simulink library "cntrlPosNdi_lib"  (R2018b)
settings: Solver=VariableStepAuto  StartTime=0.0  StopTime=10.0  RelTol=1e-3
undefined symbols (not defined in the file or in its folder): DiscIntNeverNeededParam, psc
libraries: simulink x2, $bdroot x2
settings Model: Creator=Ybeyer  LastModifiedBy=yannic
settings SFSimCC: SimUseLocalCustomCode=off
settings RTWCC: RTWUseLocalCustomCode=off
settings CodeAppCC: StateflowObjectComments=on

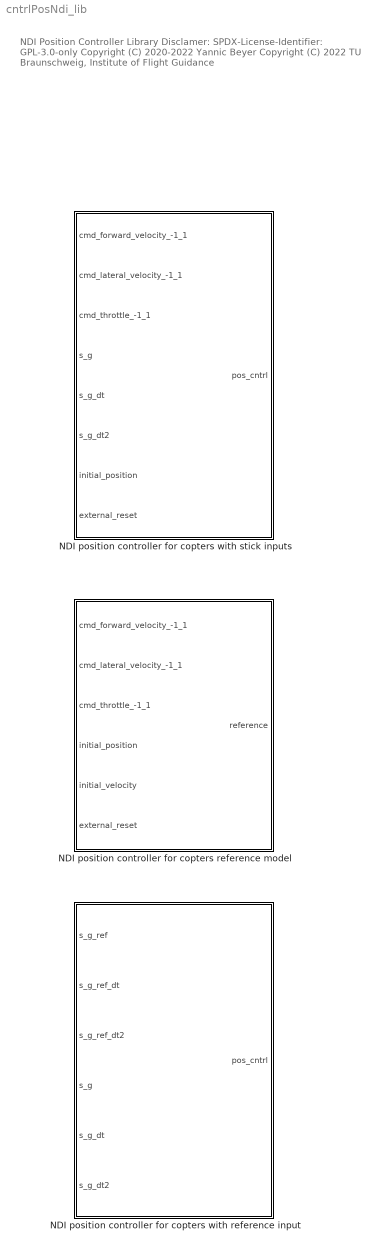
== system cntrlPosNdi_lib ==
  note: NDI Position Controller Library
      |
      | Disclamer:
      | SPDX-License-Identifier: GPL-3.0-only
      |
      | Copyright (C) 2020-2022 Yannic Beyer
      | Copyright (C) 2022 TU Braunschweig, Institute of Flight Guidance
  NDI position controller for copters reference model : Subsystem  mask{psc=psc, is_enable_checked=off, states_when_enabling=held}
      mask prompts: psc "position controller parameters struct, see cntrlPosIndi_params_default"; is_enable_checked "Activate "Enabled Subsystem""; states_when_enabling "States when enabling:"
      mask init:
      | cntrlBlockInit(is_enable_checked,states_when_enabling);
      mask TypeOptions states_when_enabling: held | reset
      mask DialogControl DescGroupVar Prompt: NDI position controller for copters reference model
      mask DialogControl DescTextVar Prompt: The commanded velocity is filtered and reference signals are generated.
  NDI position controller for copters with reference input : Subsystem  mask{psc=psc, T_inner_loop=0.1, is_enable_checked=off, states_when_enabling=held}
      mask prompts: psc "Position controller parameters struct, see cntrlPosIndi_params_default"; T_inner_loop "Inner loop time constant, in s"; is_enable_checked "Activate "Enabled Subsystem""; states_when_enabling "States when enabling:"
      mask init:
      | cntrlBlockInit(is_enable_checked,states_when_enabling);
      mask TypeOptions states_when_enabling: held | reset
      mask DialogControl DescGroupVar Prompt: NDI position controller cascade with reference inputs
      mask DialogControl DescTextVar Prompt: The controller takes reference signals as input and the control error is converted into desired accerlations.
  NDI position controller for copters with stick inputs : Subsystem  mask{psc=psc, T_inner_loop=0.1, is_enable_checked=off, states_when_enabling=held}
      mask prompts: psc "position controller parameters struct, see cntrlPosIndi_params_default"; T_inner_loop "inner loop time constant, in s"; is_enable_checked "Activate "Enabled Subsystem""; states_when_enabling "States when enabling:"
      mask init:
      | cntrlBlockInit(is_enable_checked,states_when_enabling);
      mask TypeOptions states_when_enabling: held | reset
      mask DialogControl DescGroupVar Prompt: NDI Position controller cascade
      mask DialogControl DescTextVar Prompt: The commanded velocity is filtered and the control error is converted into desired accerlations.

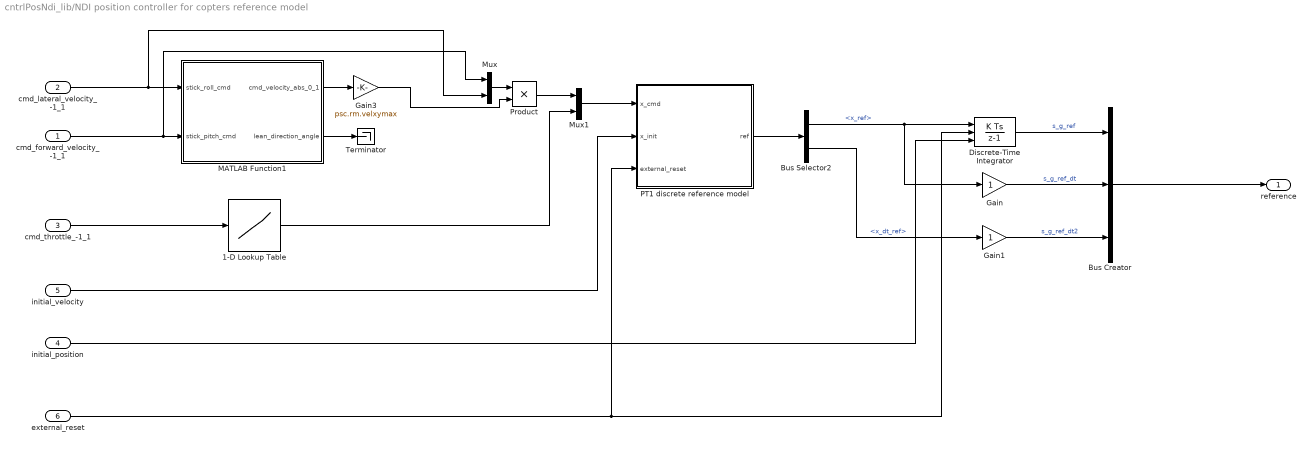
== system cntrlPosNdi_lib/NDI position controller for copters reference model ==
  cmd_forward_velocity_-1_1 : Inport
  cmd_lateral_velocity_-1_1 : Inport  Port=2
  cmd_throttle_-1_1 : Inport  Port=3
  initial_position : Inport  Port=4
  initial_velocity : Inport  Port=5
  external_reset : Inport  Port=6
  1-D Lookup Table : Lookup_n-D  NumberOfTableDimensions=1  BreakpointsForDimension1=[-1,0,1]  Table=[psc.rm.veldmax,0,-psc.rm.velumax]  InternalRulePriority=Speed  RndMeth=Simplest  InputSameDT=on
  Bus Creator : BusCreator  Inputs=3
  Bus Selector2 : BusSelector  OutputSignals=x_ref,x_dt_ref
  Discrete-Time Integrator : DiscreteIntegrator  ExternalReset=rising  InitialConditionSource=external  SampleTime=-1  ICPrevOutput=DiscIntNeverNeededParam  ICPrevScaledInput=DiscIntNeverNeededParam
  Gain : Gain
  Gain1 : Gain
  Gain3 : Gain  Gain=psc.rm.velxymax
  MATLAB Function1 : MATLAB Function  TreatAsAtomicUnit=on
  Mux : Mux  Inputs=2
  Mux1 : Mux  Inputs=2
  PT1 discrete reference model : Subsystem  mask{T=psc.rm.veltc, x_max=inf, x_min=-inf, x_dt_max=[psc.rm.accxymax*[1;1]; psc.rm.accdmax], x_dt_min=[-psc.rm.accxymax*[1;1]; -psc.rm.accumax], x_init=0}
      mask prompts: T "Time constant"; x_max "Maximum position"; x_min "Minimum position"; x_dt_max "Maximum rate"; x_dt_min "Minimum rate"; x_init "Initial position"
  Product : Product
  Terminator : Terminator
  reference : Outport
  wires:
  cmd_forward_velocity_-1_1/1 -> Mux/1, MATLAB Function1/2(stick_pitch_cmd)
  Bus Creator/1 -> reference/1
  PT1 discrete reference model/1(ref) -> Bus Selector2/1
  Discrete-Time Integrator/1 -> Bus Creator/1  "s_g_ref"
  Bus Selector2/1 -> Gain/1, Discrete-Time Integrator/1  "<x_ref>"
  Bus Selector2/2 -> Gain1/1  "<x_dt_ref>"
  cmd_lateral_velocity_-1_1/1 -> Mux/2, MATLAB Function1/1(stick_roll_cmd)
  Gain/1 -> Bus Creator/2  "s_g_ref_dt"
  Gain1/1 -> Bus Creator/3  "s_g_ref_dt2"
  Mux/1 -> Product/1
  MATLAB Function1/2(lean_direction_angle) -> Terminator/1
  MATLAB Function1/1(cmd_velocity_abs_0_1) -> Gain3/1
  Product/1 -> Mux1/1
  Gain3/1 -> Product/2
  cmd_throttle_-1_1/1 -> 1-D Lookup Table/1
  Mux1/1 -> PT1 discrete reference model/1(x_cmd)
  1-D Lookup Table/1 -> Mux1/2
  external_reset/1 -> PT1 discrete reference model/3(external_reset), Discrete-Time Integrator/2
  initial_position/1 -> Discrete-Time Integrator/3
  initial_velocity/1 -> PT1 discrete reference model/2(x_init)

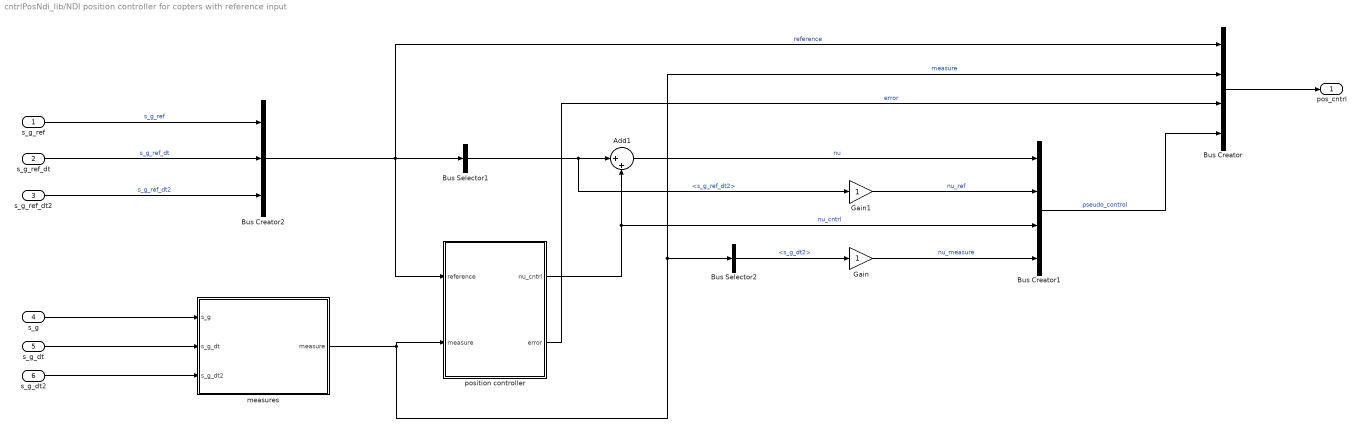
== system cntrlPosNdi_lib/NDI position controller for copters with reference input ==
  s_g_ref : Inport
  s_g_ref_dt : Inport  Port=2
  s_g_ref_dt2 : Inport  Port=3
  s_g : Inport  Port=4
  s_g_dt : Inport  Port=5
  s_g_dt2 : Inport  Port=6
  Add1 : Sum  Inputs=|++
  Bus Creator : BusCreator  Inputs=4
  Bus Creator1 : BusCreator  Inputs=4
  Bus Creator2 : BusCreator  Inputs=3
  Bus Selector1 : BusSelector  OutputSignals=s_g_ref_dt2
  Bus Selector2 : BusSelector  OutputSignals=s_g_dt2
  Gain : Gain
  Gain1 : Gain
  measures : Subsystem
  position controller : Subsystem
  pos_cntrl : Outport
  wires:
  Bus Creator2/1 -> Bus Creator/1, position controller/1(reference), Bus Selector1/1  "reference"
  position controller/1(nu_cntrl) -> Add1/2, Bus Creator1/3  "nu_cntrl"
  Add1/1 -> Bus Creator1/1  "nu"
  s_g_dt2/1 -> measures/3(s_g_dt2)
  position controller/2(error) -> Bus Creator/3  "error"
  s_g/1 -> measures/1(s_g)
  s_g_dt/1 -> measures/2(s_g_dt)
  measures/1(measure) -> position controller/2(measure), Bus Selector2/1, Bus Creator/2  "measure"
  Bus Creator1/1 -> Bus Creator/4  "pseudo_control"
  Bus Creator/1 -> pos_cntrl/1
  Gain/1 -> Bus Creator1/4  "nu_measure"
  Bus Selector1/1 -> Gain1/1, Add1/1  "<s_g_ref_dt2>"
  Gain1/1 -> Bus Creator1/2  "nu_ref"
  s_g_ref/1 -> Bus Creator2/1  "s_g_ref"
  s_g_ref_dt/1 -> Bus Creator2/2  "s_g_ref_dt"
  s_g_ref_dt2/1 -> Bus Creator2/3  "s_g_ref_dt2"
  Bus Selector2/1 -> Gain/1  "<s_g_dt2>"

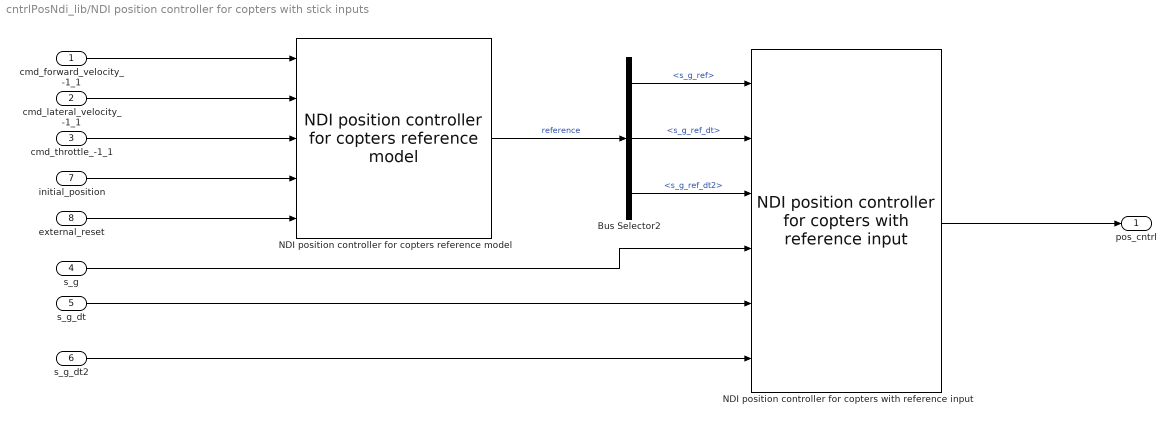
== system cntrlPosNdi_lib/NDI position controller for copters with stick inputs ==
  cmd_forward_velocity_-1_1 : Inport
  cmd_lateral_velocity_-1_1 : Inport  Port=2
  cmd_throttle_-1_1 : Inport  Port=3
  s_g : Inport  Port=4
  s_g_dt : Inport  Port=5
  s_g_dt2 : Inport  Port=6
  initial_position : Inport  Port=7
  external_reset : Inport  Port=8
  Bus Selector2 : BusSelector  OutputSignals=s_g_ref,s_g_ref_dt,s_g_ref_dt2
  NDI position controller for copters reference model : $bdroot/NDI position controller for copters reference model  psc=psc  is_enable_checked=off  states_when_enabling=held
  NDI position controller for copters with reference input : $bdroot/NDI position controller for copters with reference input  psc=psc  T_inner_loop=T_inner_loop  is_enable_checked=off  states_when_enabling=held
  pos_cntrl : Outport
  wires:
  cmd_forward_velocity_-1_1/1 -> NDI position controller for copters reference model/1
  initial_position/1 -> NDI position controller for copters reference model/4
  s_g_dt2/1 -> NDI position controller for copters with reference input/6
  s_g/1 -> NDI position controller for copters with reference input/4
  s_g_dt/1 -> NDI position controller for copters with reference input/5
  cmd_lateral_velocity_-1_1/1 -> NDI position controller for copters reference model/2
  cmd_throttle_-1_1/1 -> NDI position controller for copters reference model/3
  NDI position controller for copters reference model/1 -> Bus Selector2/1  "reference"
  Bus Selector2/1 -> NDI position controller for copters with reference input/1  "<s_g_ref>"
  Bus Selector2/2 -> NDI position controller for copters with reference input/2  "<s_g_ref_dt>"
  Bus Selector2/3 -> NDI position controller for copters with reference input/3  "<s_g_ref_dt2>"
  NDI position controller for copters with reference input/1 -> pos_cntrl/1
  external_reset/1 -> NDI position controller for copters reference model/5

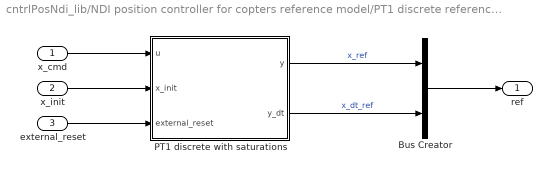
== system cntrlPosNdi_lib/NDI position controller for copters reference model/PT1 discrete reference model ==
  x_cmd : Inport
  x_init : Inport  Port=2
  external_reset : Inport  Port=3
  Bus Creator : BusCreator  Inputs=2
  PT1 discrete with saturations : Subsystem  mask{T=T, x_max=x_max, x_min=x_min, x_dt_max=x_dt_max, x_dt_min=x_dt_min, x_init=x_init}
      mask prompts: T "Time constant"; x_max "Maximum output"; x_min "Minimum output"; x_dt_max "Maximum output rate"; x_dt_min "Minimum output rate"; x_init "Initial output"
  ref : Outport
  wires:
  x_cmd/1 -> PT1 discrete with saturations/1(u)
  Bus Creator/1 -> ref/1
  PT1 discrete with saturations/1(y) -> Bus Creator/1  "x_ref"
  PT1 discrete with saturations/2(y_dt) -> Bus Creator/2  "x_dt_ref"
  external_reset/1 -> PT1 discrete with saturations/3(external_reset)
  x_init/1 -> PT1 discrete with saturations/2(x_init)

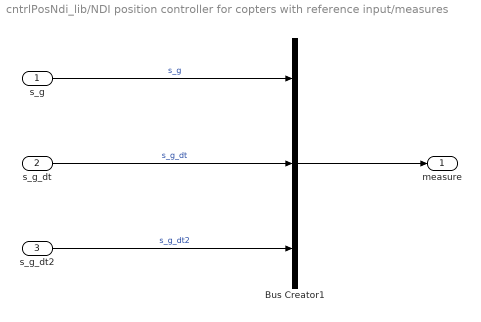
== system cntrlPosNdi_lib/NDI position controller for copters with reference input/measures ==
  s_g : Inport
  s_g_dt : Inport  Port=2
  s_g_dt2 : Inport  Port=3
  Bus Creator1 : BusCreator  Inputs=3
  measure : Outport
  wires:
  Bus Creator1/1 -> measure/1
  s_g_dt2/1 -> Bus Creator1/3  "s_g_dt2"
  s_g/1 -> Bus Creator1/1  "s_g"
  s_g_dt/1 -> Bus Creator1/2  "s_g_dt"

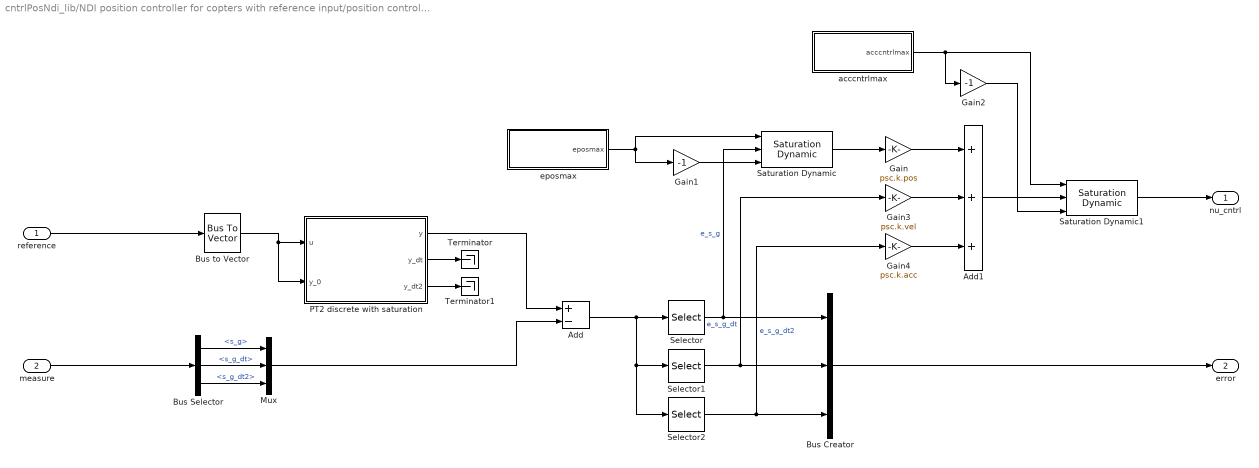
== system cntrlPosNdi_lib/NDI position controller for copters with reference input/position controller ==
  reference : Inport
  measure : Inport  Port=2
  Add : Sum  Inputs=+-
  Add1 : Sum  Inputs=+++
  Bus Creator : BusCreator  Inputs=3
  Bus Selector : BusSelector  OutputSignals=s_g,s_g_dt,s_g_dt2
  Bus to Vector : BusToVector
  Gain : Gain  Gain=psc.k.pos
  Gain1 : Gain  Gain=-1
  Gain2 : Gain  Gain=-1
  Gain3 : Gain  Gain=psc.k.vel
  Gain4 : Gain  Gain=psc.k.acc
  Mux : Mux  Inputs=3
  PT2 discrete with saturation : Subsystem  mask{omega=2./T_inner_loop, d=1, x_dt2_max=inf, x_dt2_min=-inf, x_dt_max=inf, x_dt_min=-inf, x_max=inf, x_min=-inf, x_init=0, x_dt_init=0}
      mask prompts: omega "Natural frequency"; d "Damping ratio"; x_dt2_max "Maximum acceleration"; x_dt2_min "Minimum acceleration"; x_dt_max "Maximum rate"; x_dt_min "Minimum rate"; x_max "Maximum position"; x_min "Minimum position"; x_init "Initial position"; x_dt_init "Initial rate"
  Saturation Dynamic : simulink/Discontinuities/Saturation Dynamic  OutMin=[]  OutMax=[]  OutDataTypeStr=Inherit: Same as second input  OutDataType=fixdt(1, 16)  OutScaling=2^-10  DoSatur=off
  Saturation Dynamic1 : simulink/Discontinuities/Saturation Dynamic  OutMin=[]  OutMax=[]  OutDataTypeStr=Inherit: Same as second input  OutDataType=fixdt(1, 16)  OutScaling=2^-10  DoSatur=off
  Selector : Selector  InputPortWidth=9  IndexOptions=Index vector (dialog)  Indices=1:3  OutputSizes=1
  Selector1 : Selector  InputPortWidth=9  IndexOptions=Index vector (dialog)  Indices=4:6  OutputSizes=1
  Selector2 : Selector  InputPortWidth=9  IndexOptions=Index vector (dialog)  Indices=7:9  OutputSizes=1
  Terminator : Terminator
  Terminator1 : Terminator
  acccntrlmax : MATLAB Function  TreatAsAtomicUnit=on
  eposmax : MATLAB Function  TreatAsAtomicUnit=on
  nu_cntrl : Outport
  error : Outport  Port=2
  wires:
  reference/1 -> Bus to Vector/1
  Add/1 -> Selector2/1, Selector1/1, Selector/1
  Saturation Dynamic1/1 -> nu_cntrl/1
  Add1/1 -> Saturation Dynamic1/2
  measure/1 -> Bus Selector/1
  Mux/1 -> Add/2
  Bus Selector/3 -> Mux/3  "<s_g_dt2>"
  Bus Selector/2 -> Mux/2  "<s_g_dt>"
  Bus Selector/1 -> Mux/1  "<s_g>"
  Bus to Vector/1 -> PT2 discrete with saturation/2(y_0), PT2 discrete with saturation/1(u)
  PT2 discrete with saturation/2(y_dt) -> Terminator/1
  PT2 discrete with saturation/3(y_dt2) -> Terminator1/1
  PT2 discrete with saturation/1(y) -> Add/1
  Selector/1 -> Saturation Dynamic/2, Bus Creator/1  "e_s_g"
  Selector1/1 -> Bus Creator/2, Gain3/1  "e_s_g_dt"
  Selector2/1 -> Gain4/1, Bus Creator/3  "e_s_g_dt2"
  Bus Creator/1 -> error/1
  eposmax/1(eposmax) -> Saturation Dynamic/1, Gain1/1
  Gain1/1 -> Saturation Dynamic/3
  acccntrlmax/1(acccntrlmax) -> Saturation Dynamic1/1, Gain2/1
  Gain2/1 -> Saturation Dynamic1/3
  Gain/1 -> Add1/1
  Gain3/1 -> Add1/2
  Gain4/1 -> Add1/3
  Saturation Dynamic/1 -> Gain/1

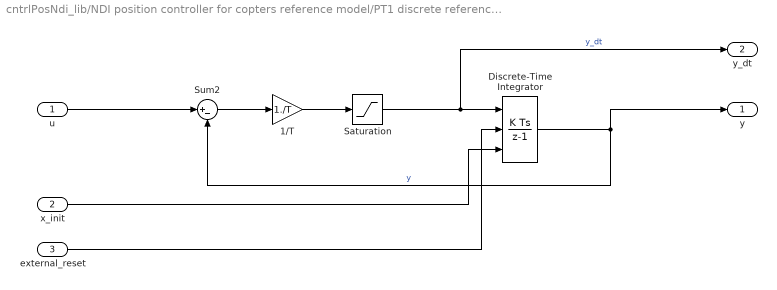
== system cntrlPosNdi_lib/NDI position controller for copters reference model/PT1 discrete reference model/PT1 discrete with saturations ==
  u : Inport
  x_init : Inport  Port=2
  external_reset : Inport  Port=3
  1/T : Gain  Gain=1./T
  Discrete-Time Integrator : DiscreteIntegrator  ExternalReset=rising  InitialConditionSource=external  InitialCondition=x_init  SampleTime=-1  LimitOutput=on  UpperSaturationLimit=x_max  LowerSaturationLimit=x_min  ICPrevOutput=DiscIntNeverNeededParam  ICPrevScaledInput=DiscIntNeverNeededParam
  Saturation : Saturate  UpperLimit=x_dt_max  LowerLimit=x_dt_min
  Sum2 : Sum  Inputs=|+-
  y : Outport
  y_dt : Outport  Port=2
  wires:
  1/T/1 -> Saturation/1
  u/1 -> Sum2/1
  Sum2/1 -> 1/T/1
  Discrete-Time Integrator/1 -> y/1, Sum2/2  "y"
  Saturation/1 -> Discrete-Time Integrator/1, y_dt/1  "y_dt"
  external_reset/1 -> Discrete-Time Integrator/2
  x_init/1 -> Discrete-Time Integrator/3

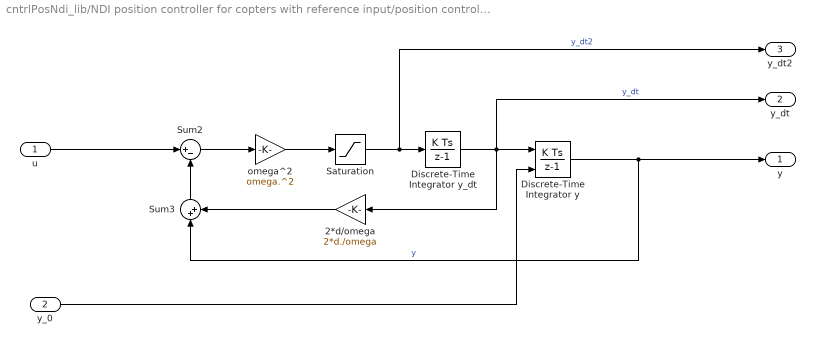
== system cntrlPosNdi_lib/NDI position controller for copters with reference input/position controller/PT2 discrete with saturation ==
  u : Inport
  y_0 : Inport  Port=2
  2*d/omega : Gain  Gain=2*d./omega
  Discrete-Time Integrator y : DiscreteIntegrator  InitialConditionSource=external  InitialCondition=x_init  SampleTime=-1  LimitOutput=on  UpperSaturationLimit=x_max  LowerSaturationLimit=x_min  ICPrevOutput=DiscIntNeverNeededParam  ICPrevScaledInput=DiscIntNeverNeededParam
  Discrete-Time Integrator y_dt : DiscreteIntegrator  InitialCondition=x_dt_init  SampleTime=-1  LimitOutput=on  UpperSaturationLimit=x_dt_max  LowerSaturationLimit=x_dt_min  ICPrevOutput=DiscIntNeverNeededParam  ICPrevScaledInput=DiscIntNeverNeededParam
  Saturation : Saturate  UpperLimit=x_dt2_max  LowerLimit=x_dt2_min
  Sum2 : Sum  Inputs=|+-
  Sum3 : Sum  Inputs=|++
  omega^2 : Gain  Gain=omega.^2
  y : Outport
  y_dt : Outport  Port=2
  y_dt2 : Outport  Port=3
  wires:
  Saturation/1 -> y_dt2/1, Discrete-Time Integrator y_dt/1  "y_dt2"
  omega^2/1 -> Saturation/1
  Sum3/1 -> Sum2/2
  u/1 -> Sum2/1
  2*d/omega/1 -> Sum3/2
  Sum2/1 -> omega^2/1
  Discrete-Time Integrator y/1 -> Sum3/1, y/1  "y"
  Discrete-Time Integrator y_dt/1 -> 2*d/omega/1, y_dt/1, Discrete-Time Integrator y/1  "y_dt"
  y_0/1 -> Discrete-Time Integrator y/2

== matlab function cntrlPosNdi_lib/NDI position controller for copters reference model/MATLAB Function1 ==
  data: stick_roll_cmd input; cmd_velocity_abs_0_1 output; stick_pitch_cmd input; lean_direction_angle output
function [cmd_velocity_abs_0_1,lean_direction_angle] = fcn(stick_roll_cmd,stick_pitch_cmd)

lean_direction_angle = atan2(stick_roll_cmd,-stick_pitch_cmd);
cmd_velocity_abs_0_1 = sqrt( stick_roll_cmd^2 + stick_pitch_cmd^2 );

end

== matlab function cntrlPosNdi_lib/NDI position controller for copters with reference input/position controller/eposmax ==
  data: eposmax output; psc parameter
function eposmax = fcn(psc)
eposmax = abs( divideFinite( psc.k.vel * psc.rm.velxymax * 0.7, psc.k.pos ) );
end

== matlab function cntrlPosNdi_lib/NDI position controller for copters with reference input/position controller/acccntrlmax ==
  data: acccntrlmax output; psc parameter
function acccntrlmax = fcn(psc)
acccntrlmax = abs( 0.75 * psc.rm.accxymax );
end
